simulink model "svpwm_inverter_model.slx"  (R2026b)
settings: Solver=VariableStepAuto  StopTime=0.02
undefined symbols (not defined in the file): L_carga, T_pwm, V_pico, Vs, Z_carga
libraries: nesl_utility x9, ee_lib x8, fl_lib x3, simulink x1
settings Model: Creator=Lemão Som  LastModifiedBy=Lemão Som
settings SimscapeCC: SimscapeLogType=all  SimscapeNominalValues="[{\"value\":\"1\",\"unit\":\"A\"},{\"value\":\"1\",\"unit\":\"bar\"},{\"value\":\"1\",\"unit\":\"cm^2\"},{\"value\":\"1\",\"unit\":\"cm^3/s\"},{\"value\":\"1\",\"unit\":\"kJ/kg\"},{\"value\":\"1\",\"unit\":\"kW\"},{\"value\":\"1\",\"unit\":\"l\"},{\"value\":\"1\",\"unit\":\"N\"},{\"value\":\"1\",\"unit\":\"N*m\"},{\"value\":\"1\",\"unit\":\"V\"},{\"value\":\"0.001\",\"unit\":\"Wb\"}]"  SimscapeUseEnergyAccounting=off

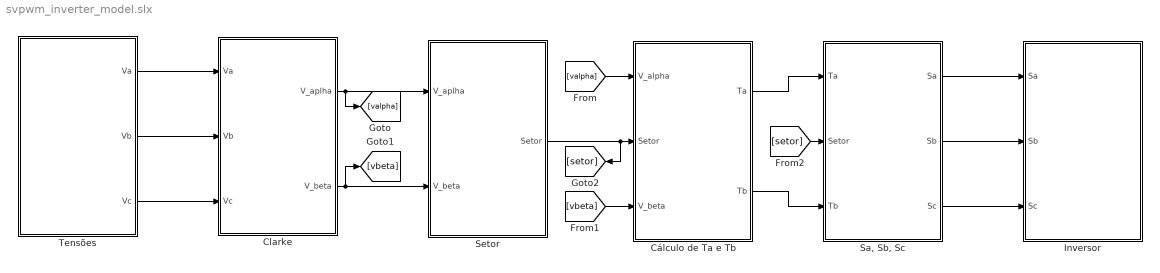
== system svpwm_inverter_model.slx ==
  Clarke : Subsystem  TreatAsAtomicUnit=on
  Cálculo de Ta e Tb : Subsystem  TreatAsAtomicUnit=on
  Inversor : Subsystem  TreatAsAtomicUnit=on
  "Sa, Sb, Sc" : Subsystem  TreatAsAtomicUnit=on
  Setor : Subsystem  TreatAsAtomicUnit=on
  Tensões : Subsystem  TreatAsAtomicUnit=on
  wires:
  Tensões/2(Vb) -> Clarke/2(Vb)
  Tensões/1(Va) -> Clarke/1(Va)
  Cálculo de Ta e Tb/1(Ta) -> "Sa, Sb, Sc"/1(Ta)
  "Sa, Sb, Sc"/3(Sc) -> Inversor/3(Sc)
  "Sa, Sb, Sc"/1(Sa) -> Inversor/1(Sa)
  Clarke/1(V_aplha) -> Setor/1(V_aplha), [valpha]
  [vbeta] -> Cálculo de Ta e Tb/3(V_beta)
  Setor/1(Setor) -> Cálculo de Ta e Tb/2(Setor), [setor]
  "Sa, Sb, Sc"/2(Sb) -> Inversor/2(Sb)
  [valpha] -> Cálculo de Ta e Tb/1(V_alpha)
  Cálculo de Ta e Tb/2(Tb) -> "Sa, Sb, Sc"/3(Tb)
  [setor] -> "Sa, Sb, Sc"/2(Setor)
  Tensões/3(Vc) -> Clarke/3(Vc)
  Clarke/2(V_beta) -> [vbeta], Setor/2(V_beta)

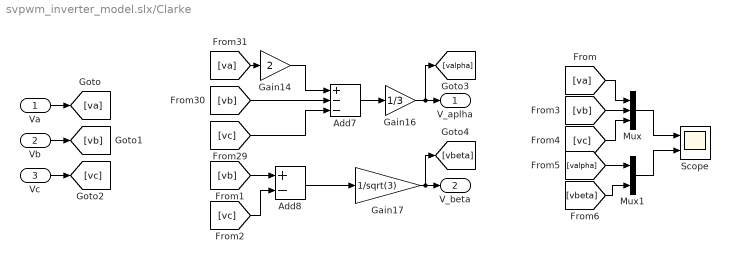
== system svpwm_inverter_model.slx/Clarke ==
  Va : Inport
  Vb : Inport  Port=2
  Vc : Inport  Port=3
  Add7 : Sum  Inputs=+--
  Add8 : Sum  Inputs=+-
  Gain14 : Gain  Gain=2
  Gain16 : Gain  Gain=1/3
  Gain17 : Gain  Gain=1/sqrt(3)
  Mux : Mux  Inputs=3
  Mux1 : Mux  Inputs=2
  Scope : Scope  NumInputPorts=2
      settings: ActiveDisplayYMinimum=-112.5  ActiveDisplayYMaximum=112.5  DataLoggingVariableName=ScopeData4
  V_aplha : Outport
  V_beta : Outport  Port=2
  wires:
  Add8/1 -> Gain17/1
  [vc] -> Add8/2
  Gain14/1 -> Add7/1
  [vb] -> Add7/2
  [vb] -> Add8/1
  Add7/1 -> Gain16/1
  [vc] -> Add7/3
  [va] -> Gain14/1
  Va/1 -> [va]
  Vb/1 -> [vb]
  Vc/1 -> [vc]
  Gain16/1 -> [valpha], V_aplha/1
  Gain17/1 -> [vbeta], V_beta/1
  [va] -> Mux/1
  [vb] -> Mux/2
  [vc] -> Mux/3
  Mux/1 -> Scope/1
  Mux1/1 -> Scope/2
  [valpha] -> Mux1/1
  [vbeta] -> Mux1/2

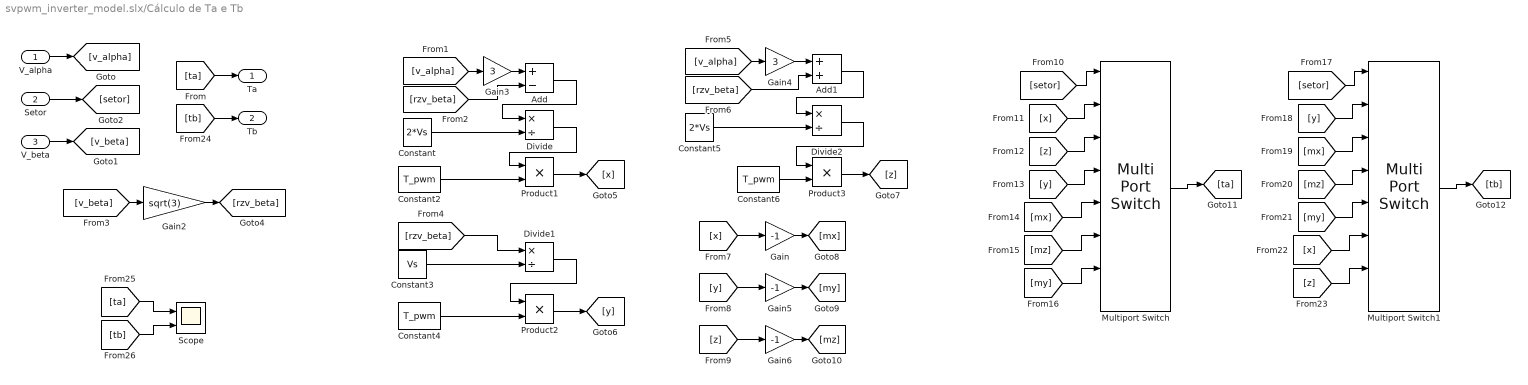
== system svpwm_inverter_model.slx/Cálculo de Ta e Tb ==
  V_alpha : Inport
  Setor : Inport  Port=2
  V_beta : Inport  Port=3
  Add : Sum  Inputs=+-
  Add1 : Sum
  Constant : Constant  Value=2*Vs  VectorParams1D=off
  Constant2 : Constant  Value=T_pwm
  Constant3 : Constant  Value=Vs
  Constant4 : Constant  Value=T_pwm
  Constant5 : Constant  Value=2*Vs
  Constant6 : Constant  Value=T_pwm
  Divide : Product  Inputs=*/
  Divide1 : Product  Inputs=*/
  Divide2 : Product  Inputs=*/
  Gain : Gain  Gain=-1
  Gain2 : Gain  Gain=sqrt(3)
  Gain3 : Gain  Gain=3
  Gain4 : Gain  Gain=3
  Gain5 : Gain  Gain=-1
  Gain6 : Gain  Gain=-1
  Multiport Switch : MultiPortSwitch  Inputs=6  DataPortForDefault=Additional data port  DiagnosticForDefault=None  SaturateOnIntegerOverflow=off  InputSameDT=off
  Multiport Switch1 : MultiPortSwitch  Inputs=6  DataPortForDefault=Additional data port  DiagnosticForDefault=None  SaturateOnIntegerOverflow=off  InputSameDT=off
  Product1 : Product
  Product2 : Product
  Product3 : Product
  Scope : Scope  NumInputPorts=2
      settings: ActiveDisplayYMinimum=-1.0546874999999907E-5  ActiveDisplayYMaximum=9.4921875000000022E-5  DataLoggingVariableName=ScopeData6
  Ta : Outport
  Tb : Outport  Port=2
  wires:
  Constant/1 -> Divide/2
  Gain2/1 -> [rzv_beta]
  [v_beta] -> Gain2/1
  V_alpha/1 -> [v_alpha]
  V_beta/1 -> [v_beta]
  Setor/1 -> [setor]
  [v_alpha] -> Gain3/1
  Gain3/1 -> Add/1
  [rzv_beta] -> Add/2
  Add/1 -> Divide/1
  Constant2/1 -> Product1/2
  Divide/1 -> Product1/1
  Product1/1 -> [x]
  Product2/1 -> [y]
  Divide1/1 -> Product2/1
  Constant4/1 -> Product2/2
  Constant3/1 -> Divide1/2
  [rzv_beta] -> Divide1/1
  Product3/1 -> [z]
  Divide2/1 -> Product3/1
  Constant6/1 -> Product3/2
  Add1/1 -> Divide2/1
  [rzv_beta] -> Add1/2
  Gain4/1 -> Add1/1
  [v_alpha] -> Gain4/1
  Constant5/1 -> Divide2/2
  [x] -> Gain/1
  [y] -> Gain5/1
  [z] -> Gain6/1
  Gain/1 -> [mx]
  Gain5/1 -> [my]
  Gain6/1 -> [mz]
  [setor] -> Multiport Switch/1
  [x] -> Multiport Switch/2
  [z] -> Multiport Switch/3
  [y] -> Multiport Switch/4
  [mx] -> Multiport Switch/5
  [mz] -> Multiport Switch/6
  [my] -> Multiport Switch/7
  Multiport Switch/1 -> [ta]
  Multiport Switch1/1 -> [tb]
  [z] -> Multiport Switch1/7
  [x] -> Multiport Switch1/6
  [my] -> Multiport Switch1/5
  [mz] -> Multiport Switch1/4
  [mx] -> Multiport Switch1/3
  [y] -> Multiport Switch1/2
  [setor] -> Multiport Switch1/1
  [ta] -> Ta/1
  [tb] -> Tb/1
  [ta] -> Scope/1
  [tb] -> Scope/2

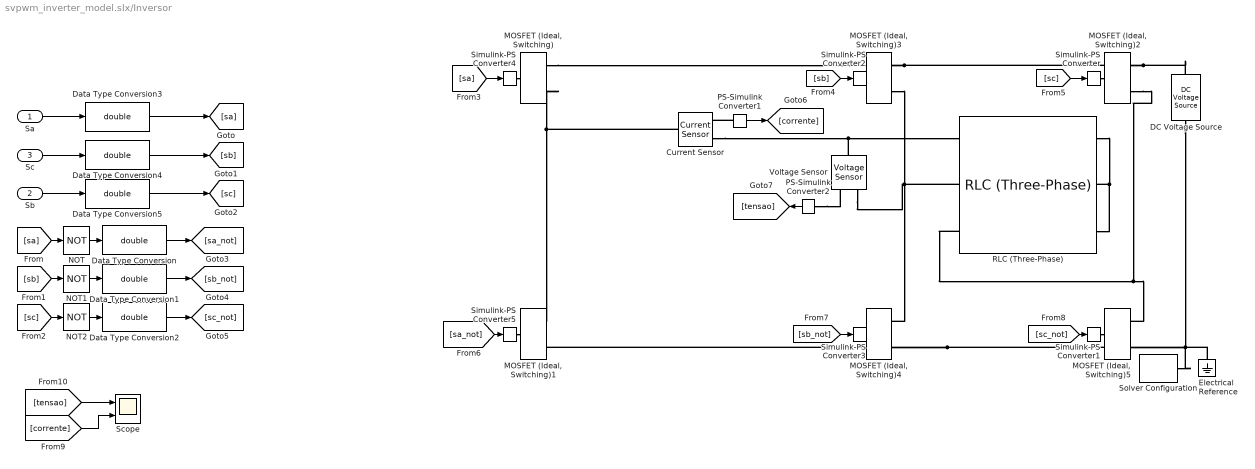
== system svpwm_inverter_model.slx/Inversor ==
  Sa : Inport
  Sb : Inport  Port=2
  Sc : Inport  Port=3
  Current Sensor : fl_lib/Electrical/Electrical Sensors/Current Sensor
  DC Voltage Source : ee_lib/Additional Components/SPICE Sources/DC Voltage Source  DC=160 V
  Data Type Conversion{,1..5} (6 alike) : DataTypeConversion  OutDataTypeStr=double  SaturateOnIntegerOverflow=off  RndMeth=Floor
  Electrical Reference : fl_lib/Electrical/Electrical Elements/Electrical Reference
  MOSFET (Ideal, Switching){,1..5} (6 alike) : ee_lib/Semiconductors & Converters/MOSFET (Ideal, Switching)  port_option=ee.enum.controlport.ps  Rds=0.01 Ohm  Goff=1e-6 1/Ohm  Vth=0.5 V  diode_param=ee.enum.semiconductors.protectionDiode.nodynamics  diode_Vf=0.8 V  diode_Ron=0.001 Ohm  diode_Goff=1e-5 1/Ohm  diode_C=50e-9 F  diode_iRM=-235 A  diode_iF=300 A  diode_idot=-50 A/us  diode_trr_param=ee.enum.converters.diodeReverseParam.trr_factor  diode_trr_factor=3  diode_trr=15 us  diode_Qrr=1500 s*uA  ids_specify=off  ids_priority=None  ids=0 A  ids_nominal_specify=off  ids_nominal_value=1  ids_nominal_unit=A  vds_specify=off  vds_priority=None  vds=0 V  vds_nominal_specify=off  vds_nominal_value=1  vds_nominal_unit=V  vgs_specify=off  vgs_priority=None  vgs=0 V  vgs_nominal_specify=off  vgs_nominal_value=1  vgs_nominal_unit=V  thermal_loss_option=ee.enum.converters.thermalLossOption.constantvalues  Von_data=[0, 1.8, 3.2, 6, 10, 16; 0, 2, 5.5, 9.5, 15, 25] V  Tj=[298.15, 448.15] K  Iout_data=[0, 20, 40, 60, 80, 100] A  tabulateWithVds=false  Eon_data=[0, 55.04, 124.57, 235.53, 362.12; 0, 71.25, 161.25, 304.88, 468.75] * 1e-6 J  Eoff_data=[0, 18, 30, 56.1, 76.5; 0, 22.5, 37.5, 70.13, 95.63] * 1e-6 J  Eon_data_3D=[zeros(2, 5, 3)] J  Eoff_data_3D=[zeros(2, 5, 3)] J  Tj_loss=[298.15, 448.15] K  Iout_data_loss=[0, 10, 20, 30, 40] A  Vds_loss=[0, 150, 300] V  Eon_scalar=22.86e-3 J  Eoff_scalar=17.14e-3 J  Voff=300 V  Iout_scalar=600 A  useCurrentFromPreviousCycle=false  currentMeasDelay=0 s  useVoltageFromPreviousCycle=false  voltageMeasDelay=0 s  diodeModelType=ee.enum.converters.diodeModelType.pwl  diodeTableType=ee.enum.diode.tableType.IfMat  diode_ReverseIVType=ee.enum.diode.diodeReverseIV.constant  diode_IfMat=[.07, .12, .19, 1.75, 4.24, 7.32, 11.2; .16, .3, .72, 2.14, 4.02, 6.35, 9.12] A  diode_VfMat=[.9, 1.15, 1.25, 1.5, 1.75, 2.17, 2.6, 2.85; .58, .68, .75, 1.1, 1.38, 1.77, 2.27, 2.7] V  diode_TjVec=[25, 125] degC  diode_VfVec=[.5, .7, .9, 1.3, 1.7, 2.1, 2.5] V  diode_IfVec=[.1, .2, .5, 1, 2, 4, 7, 10] A  diode_IrMat=[1e-06, 2e-06, 5e-06, 1e-05, 2.5e-05, 5e-05, .0001; 2e-06, 5e-06, 1e-05, 4e-05, 8e-05, .0002, .0005] A  diode_VrMat=[10, 100, 200, 250, 300, 325, 350; 10, 70, 160, 220, 270, 300, 320] V  diode_VrVec=[10, 20, 40, 50, 70, 80, 100] V  diode_IrVec=[1e-06, 2e-06, 5e-06, 1e-05, 2e-05, 5e-05, .0001] A  diode_Vr=-600 V  diode_Ls=150 nH  diode_Erec=0.03 J  diode_rec_loss_model=ee.enum.diode.reverseRecoveryModelTabulateUpTo3D.fixed  diode_ErecVal=0 J  diode_scaleWithIandV=true  diode_ErecMat=zeros(2, 3) J  diodeErecMat3D=zeros(2, 3, 2) J  diode_TjrecVec=[298.15, 398.15] K  diode_IfrecVec=[.1, 1, 10] A  diodeVrecVec=[0, 100] V  diode_IrecVal=10 A  diode_VrecVal=10 V  diode_tFilter=1 / 1000 / 100 s  separateThermalPortForDiode=false  thermal_network_parameterization=ee.enum.thermalNetworkTopology.external  Rth=[.03, .2] K/W  Rth_Cauer=[.03, .1, .2] K/W  Rth_Foster=[.08, .14, .22, .16] K/W  thermal_mass_parameterization=ee.enum.thermalNetwork.timeconstant  thermal_mass=[3, 25] J/K  thermal_mass_Cauer=[3, 10, 25] J/K  thermal_mass_Foster=[.001, .005, .05, .5] J/K  thermal_time_constant=[.1, 5] s  thermal_time_constant_Cauer=[.1, 1, 5] s  thermal_time_constant_Foster=[7e-05, .0007, .01, .08] s  thermal_mass_initial_temperatures=[25, 25] degC  thermal_mass_initial_temperatures_Cauer=[25, 25, 25] degC  junction_thermal_mass=0.1 J/K  Tvec_initial_Foster=[25, 25, 25, 25] degC  RthDiode=[.03, .2] K/W  RthCauerDiode=[.03, .1, .2] K/W  RthFosterDiode=[.03, .2] K/W  thermalMassDiode=[3, 25] J/K  thermalMassCauerDiode=[3, 10, 25] J/K  thermalMassFosterDiode=[33, 50] J/K  thermalTauDiode=[.1, 5] s  thermalTauCauerDiode=[.1, 1, 5] s  thermalTauFosterDiode=[1, 10] s  thermalMassInitTempDiode=[25, 25] degC  thermalMassInitTempCauerDiode=[25, 25, 25] degC  junctionthermalMassDiode=0.1 J/K  TVecInitialFosterDiode=[25, 25, 25, 25] degC  no_thermal_network=ee.enum.enable.no  mosfet_junction_temperature_specify=off  mosfet_junction_temperature_priority=None  mosfet_junction_temperature=25 degC  mosfet_junction_temperature_nominal_specify=off  mosfet_junction_temperature_nominal_value=1  mosfet_junction_temperature_nominal_unit=degC  diode_junction_temperature_specify=off  diode_junction_temperature_priority=None  diode_junction_temperature=25 degC  diode_junction_temperature_nominal_specify=off  diode_junction_temperature_nominal_value=1  diode_junction_temperature_nominal_unit=degC  Qj_specify=off  Qj_priority=None  Qj=0 W  Qj_nominal_specify=off  Qj_nominal_value=1  Qj_nominal_unit=W  accumulatedSwitchingLosses_specify=off  accumulatedSwitchingLosses_priority=None  accumulatedSwitchingLosses=0 J
  NOT : Logic  Operator=NOT  IconShape=distinctive  AllPortsSameDT=off  OutDataTypeStr=boolean
  NOT1 : Logic  Operator=NOT  IconShape=distinctive  AllPortsSameDT=off  OutDataTypeStr=boolean
  NOT2 : Logic  Operator=NOT  IconShape=distinctive  AllPortsSameDT=off  OutDataTypeStr=boolean
  PS-Simulink Converter1 : nesl_utility/PS-Simulink Converter  PhysicalDomain=network_engine_domain  SubClassName=ps_output  LeftPortType=input  RightPortType=output  PseudoPeriodic=off  Frequencies=[]  VectorFormat=inherit  Unit=inherit  AffineConversion=off
  PS-Simulink Converter2 : nesl_utility/PS-Simulink Converter  PhysicalDomain=network_engine_domain  SubClassName=ps_output  LeftPortType=input  RightPortType=output  PseudoPeriodic=off  Frequencies=[]  VectorFormat=inherit  Unit=inherit  AffineConversion=off
  RLC (Three-Phase) : ee_lib/Passive/RLC Assemblies/RLC (Three-Phase)  port_option=ee.enum.threePhasePort.expanded  component_structure=ee.enum.rlc.structure.SeriesRL  R=Z_carga Ohm  L=L_carga H  C=1e-6 F  R_parasitic=0 Ohm  G_parasitic=0 1/Ohm  IL_specify=off  IL_priority=High  IL=[0, 0, 0] A  IL_nominal_specify=off  IL_nominal_value=1  IL_nominal_unit=A  VC_specify=off  VC_priority=High  VC=[0, 0, 0] V  VC_nominal_specify=off  VC_nominal_value=1  VC_nominal_unit=V
  Scope : Scope  NumInputPorts=2
      settings: ActiveDisplayYMinimum=-200.03272268946458  ActiveDisplayYMaximum=200.03209581864482  DataLoggingVariableName=ScopeData2
  Simulink-PS Converter{,1..5} (6 alike) : nesl_utility/Simulink-PS Converter  PhysicalDomain=network_engine_domain  SubClassName=ps_input  LeftPortType=input  RightPortType=output  PseudoPeriodic=off  Frequencies=[]  NoiseDistribution=none  NoiseParameters=[]  Unit=1  AffineConversion=off  FilteringAndDerivatives=provide  SimscapeFilterOrder=1  InputFilterTimeConstant=0.001  UdotUserProvided=0
  Solver Configuration : nesl_utility/Solver Configuration  PhysicalDomain=network_engine_domain  SubClassName=solver  LeftPortType=input  RightPortType=generic  Tones=[]  Harmonics=[]  SimulateNoise=off  Profile=off  UseLocalSampling=off  EnableSwitchedLinearOptims=on  FrequencyDomain=off  UseCCode=off  RelTol=0.001  AbsTol=0.001  MinStep=1e-09  ToWorkspace=off  RevertToSquareIcSolve=off  NumHomotopyIterations=100  PhasorMode=off  PhasorModeNumHarmonics=1  ConsistencySolver=NEWTON_XTOL_AFTER_FTOL  CanonicalOrdering=CANONICAL  OptimizeIntermediates=OPTIMIZED  MulticoreSolverChoice=BACKWARD_EULER  IndexReductionMethod=DerivativeReplacement  DoDC=off  ResidualTolerance=1e-09  ConsistencyTolSource=LOCAL  ConsistencyAbsTol=0.001  ConsistencyRelTol=0.001  ConsistencyTolFactor=0.001  UseLocalSolver=off  LocalSolverChoice=NE_BACKWARD_EULER_ADVANCER  ResolveIndetEquations=on  FunctionEvalNumThread=1  LocalSolverSampleTime=0.001  DoFixedCost=off  MaxNonlinIter=3  MaxModeIter=2  ComputeImpulses=off  ImpulseIterations=2  LinearAlgebra=auto  LinearAlgebraNumThread=0  EquationFormulation=NE_TIME_EF  DelaysMemoryBudget=1024  AutomaticFiltering=on  FilteringTimeConstant=0.001  PartitionStorageMethod=AS_NEEDED  PartitionMemoryBudget=1024  PartitionMethod=BALANCED  MultibodyUseLocalSolver=off  MultibodyLocalSolverChoice=ODE1  MultibodyLocalSolverSampleTime=0.001
  Voltage Sensor : fl_lib/Electrical/Electrical Sensors/Voltage Sensor
  wires:
  Sb/1 -> Data Type Conversion5/1
  Sa/1 -> Data Type Conversion3/1
  Sc/1 -> Data Type Conversion4/1
  [sa] -> NOT/1
  [sb] -> NOT1/1
  [sc] -> NOT2/1
  NOT/1 -> Data Type Conversion/1
  NOT1/1 -> Data Type Conversion1/1
  NOT2/1 -> Data Type Conversion2/1
  [sc] -> Simulink-PS Converter/1
  [sc_not] -> Simulink-PS Converter1/1
  [sb] -> Simulink-PS Converter2/1
  [sb_not] -> Simulink-PS Converter3/1
  [sa] -> Simulink-PS Converter4/1
  [sa_not] -> Simulink-PS Converter5/1
  Data Type Conversion/1 -> [sa_not]
  Data Type Conversion1/1 -> [sb_not]
  Data Type Conversion2/1 -> [sc_not]
  Data Type Conversion3/1 -> [sa]
  Data Type Conversion4/1 -> [sb]
  Data Type Conversion5/1 -> [sc]
  PS-Simulink Converter1/1 -> [corrente]
  PS-Simulink Converter2/1 -> [tensao]
  [tensao] -> Scope/1
  [corrente] -> Scope/2
  connections:
  Simulink-PS Converter/RConn1 -- "MOSFET (Ideal, Switching)2"/LConn1
  Simulink-PS Converter1/RConn1 -- "MOSFET (Ideal, Switching)5"/LConn1
  Simulink-PS Converter2/RConn1 -- "MOSFET (Ideal, Switching)3"/LConn1
  Simulink-PS Converter3/RConn1 -- "MOSFET (Ideal, Switching)4"/LConn1
  Simulink-PS Converter4/RConn1 -- "MOSFET (Ideal, Switching)"/LConn1
  Simulink-PS Converter5/RConn1 -- "MOSFET (Ideal, Switching)1"/LConn1
  DC Voltage Source/RConn1 -- Solver Configuration/RConn1 -- Electrical Reference/LConn1 -- "MOSFET (Ideal, Switching)5"/RConn2 -- "MOSFET (Ideal, Switching)4"/RConn2 -- "MOSFET (Ideal, Switching)1"/RConn2
  DC Voltage Source/LConn1 -- "MOSFET (Ideal, Switching)2"/RConn1 -- "MOSFET (Ideal, Switching)"/RConn1 -- "MOSFET (Ideal, Switching)3"/RConn1
  "MOSFET (Ideal, Switching)"/RConn2 -- "MOSFET (Ideal, Switching)1"/RConn1 -- Current Sensor/LConn1
  "MOSFET (Ideal, Switching)3"/RConn2 -- RLC (Three-Phase)/LConn2 -- Voltage Sensor/RConn2 -- "MOSFET (Ideal, Switching)4"/RConn1
  RLC (Three-Phase)/RConn1 -- RLC (Three-Phase)/RConn3 -- RLC (Three-Phase)/RConn2
  RLC (Three-Phase)/LConn3 -- "MOSFET (Ideal, Switching)5"/RConn1 -- "MOSFET (Ideal, Switching)2"/RConn2
  Current Sensor/RConn2 -- Voltage Sensor/LConn1 -- RLC (Three-Phase)/LConn1
  PS-Simulink Converter1/LConn1 -- Current Sensor/RConn1
  PS-Simulink Converter2/LConn1 -- Voltage Sensor/RConn1

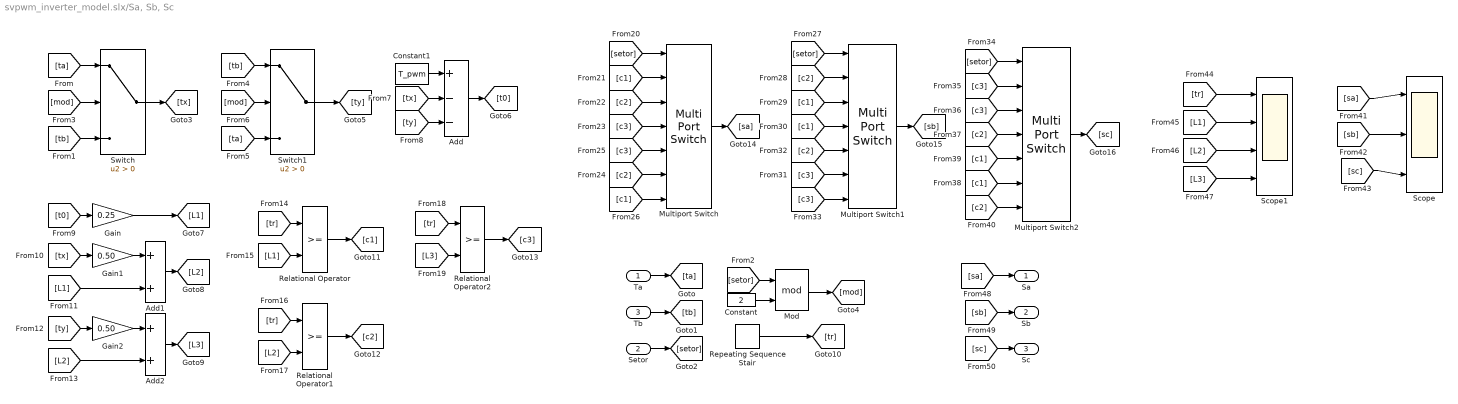
== system svpwm_inverter_model.slx/Sa, Sb, Sc ==
  Ta : Inport
  Setor : Inport  Port=2
  Tb : Inport  Port=3
  Add : Sum  Inputs=+--
  Add1 : Sum
  Add2 : Sum
  Constant : Constant  Value=2
  Constant1 : Constant  Value=T_pwm
  Gain : Gain  Gain=0.25
  Gain1 : Gain  Gain=0.50
  Gain2 : Gain  Gain=0.50
  Mod : Math  Operator=mod
  Multiport Switch : MultiPortSwitch  Inputs=6  DiagnosticForDefault=None  SaturateOnIntegerOverflow=off  InputSameDT=off
  Multiport Switch1 : MultiPortSwitch  Inputs=6  DiagnosticForDefault=None  SaturateOnIntegerOverflow=off  InputSameDT=off
  Multiport Switch2 : MultiPortSwitch  Inputs=6  DiagnosticForDefault=None  SaturateOnIntegerOverflow=off  InputSameDT=off
  Relational Operator : RelationalOperator  OutDataTypeStr=boolean  RndMeth=Simplest  InputSameDT=off
  Relational Operator1 : RelationalOperator  OutDataTypeStr=boolean  RndMeth=Simplest  InputSameDT=off
  Relational Operator2 : RelationalOperator  OutDataTypeStr=boolean  RndMeth=Simplest  InputSameDT=off
  Repeating Sequence Stair : simulink/Sources/Repeating Sequence Stair  OutValues=[linspace(0, 5e-5, 50), linspace(5e-5, 0, 50)]'  tsamp=1e-6  OutMin=[]  OutMax=[]  OutDataTypeStr=double  OutputDataTypeScalingMode=double  OutDataType=fixdt(0,8)  ConRadixGroup=Best Precision: Vector-wise  OutScaling=2^-12
  Scope : Scope  NumInputPorts=3
      settings: ActiveDisplayYMinimum=-0.12463329847231375  ActiveDisplayYMaximum=1.089767692485754
  Scope1 : Scope  NumInputPorts=4
      settings: ActiveDisplayYMinimum=-6.2499999999999986E-6  ActiveDisplayYMaximum=5.6250000000000005E-5
  Switch : Switch  Criteria=u2 > Threshold  SaturateOnIntegerOverflow=off  InputSameDT=off
  Switch1 : Switch  Criteria=u2 > Threshold  SaturateOnIntegerOverflow=off  InputSameDT=off
  Sa : Outport
  Sb : Outport  Port=2
  Sc : Outport  Port=3
  wires:
  Tb/1 -> [tb]
  Ta/1 -> [ta]
  [tb] -> Switch/3
  [ta] -> Switch/1
  Setor/1 -> [setor]
  Switch/1 -> [tx]
  [setor] -> Mod/1
  Constant/1 -> Mod/2
  Mod/1 -> [mod]
  [mod] -> Switch/2
  [mod] -> Switch1/2
  Switch1/1 -> [ty]
  [tb] -> Switch1/1
  [ta] -> Switch1/3
  Constant1/1 -> Add/1
  Add/1 -> [t0]
  [t0] -> Gain/1
  [tx] -> Gain1/1
  Gain/1 -> [L1]
  Gain1/1 -> Add1/1
  [L1] -> Add1/2
  Add1/1 -> [L2]
  Add2/1 -> [L3]
  [L2] -> Add2/2
  Gain2/1 -> Add2/1
  [ty] -> Gain2/1
  [tr] -> Relational Operator/1
  [L1] -> Relational Operator/2
  [L2] -> Relational Operator1/2
  [tr] -> Relational Operator1/1
  [tr] -> Relational Operator2/1
  [L3] -> Relational Operator2/2
  Relational Operator/1 -> [c1]
  Relational Operator1/1 -> [c2]
  Relational Operator2/1 -> [c3]
  [setor] -> Multiport Switch/1
  [c1] -> Multiport Switch/2
  [c2] -> Multiport Switch/3
  [c3] -> Multiport Switch/4
  [c2] -> Multiport Switch/6
  [c3] -> Multiport Switch/5
  [c1] -> Multiport Switch/7
  Multiport Switch/1 -> [sa]
  Multiport Switch1/1 -> [sb]
  [c3] -> Multiport Switch1/7
  [c2] -> Multiport Switch1/5
  [c3] -> Multiport Switch1/6
  [c1] -> Multiport Switch1/4
  [c1] -> Multiport Switch1/3
  [c2] -> Multiport Switch1/2
  [setor] -> Multiport Switch1/1
  [setor] -> Multiport Switch2/1
  [c3] -> Multiport Switch2/2
  [c3] -> Multiport Switch2/3
  [c2] -> Multiport Switch2/4
  [c1] -> Multiport Switch2/6
  [c1] -> Multiport Switch2/5
  [c2] -> Multiport Switch2/7
  Multiport Switch2/1 -> [sc]
  [sa] -> Scope/1
  [sb] -> Scope/2
  [sc] -> Scope/3
  [tr] -> Scope1/1
  [L1] -> Scope1/2
  [L2] -> Scope1/3
  [L3] -> Scope1/4
  Repeating Sequence Stair/1 -> [tr]
  [tx] -> Add/2
  [ty] -> Add/3
  [sa] -> Sa/1
  [sb] -> Sb/1
  [sc] -> Sc/1

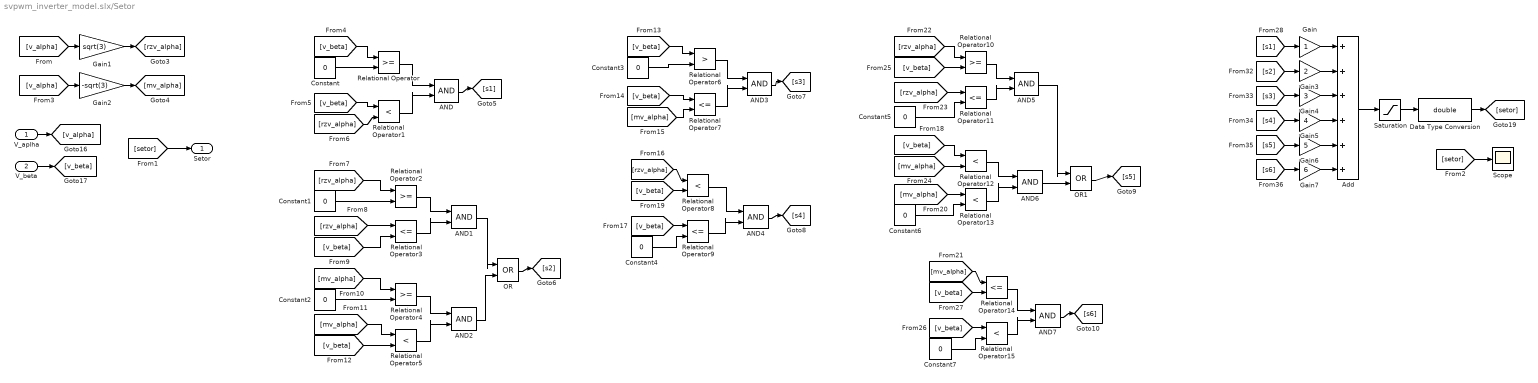
== system svpwm_inverter_model.slx/Setor ==
  V_aplha : Inport
  V_beta : Inport  Port=2
  AND{,1..7} (8 alike) : Logic  IconShape=distinctive  AllPortsSameDT=off  OutDataTypeStr=boolean
  Add : Sum  Inputs=++++++
  Constant{,1..7} (8 alike) : Constant  Value=0
  Data Type Conversion : DataTypeConversion  OutDataTypeStr=double  SaturateOnIntegerOverflow=off  RndMeth=Floor
  Gain : Gain
  Gain1 : Gain  Gain=sqrt(3)
  Gain2 : Gain  Gain=-sqrt(3)
  Gain3 : Gain  Gain=2
  Gain4 : Gain  Gain=3
  Gain5 : Gain  Gain=4
  Gain6 : Gain  Gain=5
  Gain7 : Gain  Gain=6
  OR : Logic  Operator=OR  IconShape=distinctive  AllPortsSameDT=off  OutDataTypeStr=boolean
  OR1 : Logic  Operator=OR  IconShape=distinctive  AllPortsSameDT=off  OutDataTypeStr=boolean
  Relational Operator{,2,4,10} (4 alike) : RelationalOperator  OutDataTypeStr=boolean  RndMeth=Simplest  InputSameDT=off
  Relational Operator{1,5,8,12..13,15} (6 alike) : RelationalOperator  Operator=<  OutDataTypeStr=boolean  RndMeth=Simplest  InputSameDT=off
  Relational Operator{3,7,9,11,14} (5 alike) : RelationalOperator  Operator=<=  OutDataTypeStr=boolean  RndMeth=Simplest  InputSameDT=off
  Relational Operator6 : RelationalOperator  Operator=>  OutDataTypeStr=boolean  RndMeth=Simplest  InputSameDT=off
  Saturation : Saturate  UpperLimit=6  LowerLimit=1
  Scope : Scope
      settings: ActiveDisplayYMinimum=0.37500000000000022  ActiveDisplayYMaximum=6.625  DataLoggingVariableName=ScopeData5
  Setor : Outport
  wires:
  Relational Operator13/1 -> AND6/2
  Relational Operator9/1 -> AND4/2
  Constant2/1 -> Relational Operator4/2
  [s2] -> Gain3/1
  [v_beta] -> Relational Operator14/2
  Relational Operator/1 -> AND/1
  [v_beta] -> Relational Operator10/2
  [v_beta] -> Relational Operator8/2
  [mv_alpha] -> Relational Operator7/2
  [v_beta] -> Relational Operator7/1
  Constant1/1 -> Relational Operator2/2
  Relational Operator8/1 -> AND4/1
  Relational Operator1/1 -> AND/2
  [v_beta] -> Relational Operator6/1
  [v_alpha] -> Gain2/1
  [rzv_alpha] -> Relational Operator8/1
  [mv_alpha] -> Relational Operator4/1
  [rzv_alpha] -> Relational Operator3/1
  [rzv_alpha] -> Relational Operator10/1
  Relational Operator6/1 -> AND3/1
  Relational Operator2/1 -> AND1/1
  AND3/1 -> [s3]
  Constant3/1 -> Relational Operator6/2
  Relational Operator15/1 -> AND7/2
  AND/1 -> [s1]
  [s5] -> Gain6/1
  [v_beta] -> Relational Operator3/2
  Relational Operator11/1 -> AND5/2
  Gain2/1 -> [mv_alpha]
  Gain1/1 -> [rzv_alpha]
  Relational Operator3/1 -> AND1/2
  [v_beta] -> Relational Operator9/1
  Constant/1 -> Relational Operator/2
  [v_beta] -> Relational Operator15/1
  AND4/1 -> [s4]
  [s1] -> Gain/1
  Relational Operator12/1 -> AND6/1
  [v_alpha] -> Gain1/1
  AND7/1 -> [s6]
  Relational Operator7/1 -> AND3/2
  Constant5/1 -> Relational Operator11/2
  [mv_alpha] -> Relational Operator14/1
  Relational Operator4/1 -> AND2/1
  [v_beta] -> Relational Operator1/1
  AND2/1 -> OR/2
  [s4] -> Gain5/1
  Relational Operator10/1 -> AND5/1
  [v_beta] -> Relational Operator/1
  [rzv_alpha] -> Relational Operator2/1
  [rzv_alpha] -> Relational Operator1/2
  Add/1 -> Saturation/1
  [mv_alpha] -> Relational Operator5/1
  Relational Operator14/1 -> AND7/1
  Relational Operator5/1 -> AND2/2
  [v_beta] -> Relational Operator5/2
  Constant7/1 -> Relational Operator15/2
  [s3] -> Gain4/1
  [mv_alpha] -> Relational Operator12/2
  [mv_alpha] -> Relational Operator13/1
  AND6/1 -> OR1/2
  [v_beta] -> Relational Operator12/1
  [rzv_alpha] -> Relational Operator11/1
  [s6] -> Gain7/1
  Constant6/1 -> Relational Operator13/2
  Constant4/1 -> Relational Operator9/2
  V_aplha/1 -> [v_alpha]
  V_beta/1 -> [v_beta]
  Gain/1 -> Add/1
  Gain3/1 -> Add/2
  Gain4/1 -> Add/3
  Gain5/1 -> Add/4
  Gain6/1 -> Add/5
  Gain7/1 -> Add/6
  [setor] -> Setor/1
  AND1/1 -> OR/1
  OR/1 -> [s2]
  OR1/1 -> [s5]
  AND5/1 -> OR1/1
  Data Type Conversion/1 -> [setor]
  Saturation/1 -> Data Type Conversion/1
  [setor] -> Scope/1

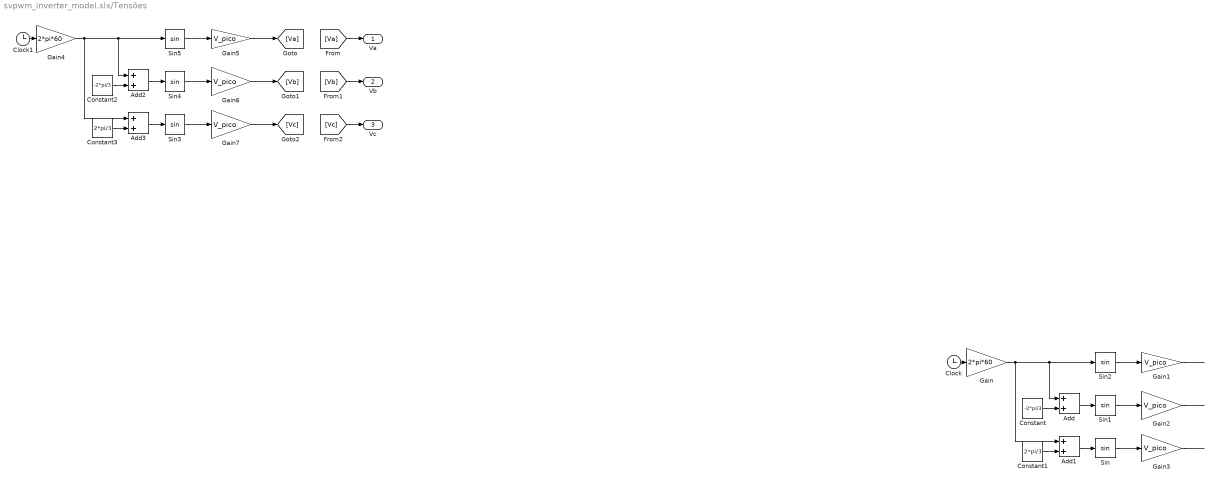
== system svpwm_inverter_model.slx/Tensões ==
  Add{,1..3} (4 alike) : Sum
  Clock : Clock
  Clock1 : Clock
  Constant : Constant  Value=-2*pi/3
  Constant1 : Constant  Value=2*pi/3
  Constant2 : Constant  Value=-2*pi/3
  Constant3 : Constant  Value=2*pi/3
  Gain : Gain  Gain=2*pi*60
  Gain{1..3,5..7} (6 alike) : Gain  Gain=V_pico
  Gain4 : Gain  Gain=2*pi*60
  Sin{,1..5} (6 alike) : Trigonometry
  Va : Outport
  Vb : Outport  Port=2
  Vc : Outport  Port=3
  wires:
  Constant1/1 -> Add1/2
  Constant/1 -> Add/2
  Add/1 -> Sin1/1
  Gain3/1 -> ?
  Gain/1 -> Add1/1, Sin2/1, Add/1
  Sin2/1 -> Gain1/1
  Add1/1 -> Sin/1
  Gain2/1 -> ?
  Sin1/1 -> Gain2/1
  Gain1/1 -> ?
  Clock/1 -> Gain/1
  Sin/1 -> Gain3/1
  Constant3/1 -> Add3/2
  Constant2/1 -> Add2/2
  Add2/1 -> Sin4/1
  Gain4/1 -> Add3/1, Sin5/1, Add2/1
  Sin5/1 -> Gain5/1
  Add3/1 -> Sin3/1
  Sin4/1 -> Gain6/1
  Clock1/1 -> Gain4/1
  Sin3/1 -> Gain7/1
  Gain5/1 -> [Va]
  Gain6/1 -> [Vb]
  Gain7/1 -> [Vc]
  [Va] -> Va/1
  [Vb] -> Vb/1
  [Vc] -> Vc/1
